simulink model "ceto"  (R2025a)
settings: Solver=ode4  StartTime=0  StopTime=200  FixedStep=0.01  MaxStep=0.01  RelTol=1e-3  EnableMultiTasking=on
values from neighbouring files (symbols this model uses):
  bemDepths = -3.0:-0.1:-15.0    [wecSimInputFile.m]
  PTO_motion_amplitude = 6    [wecSimInputFile.m]
  PTO_motion_period = 10    [createMCRMat.m]    (also in wecSimInputFile.m)
undefined symbols (not defined in the file or in its folder): body, pto
libraries: WECSim_Lib_Body_Elements x1, WECSim_Lib_Frames x1, WECSim_Lib_PTOs x1
settings Model: Creator=mlawson  LastModifiedBy=akeeste
settings SolverCC: ZeroCrossControl=DisableAll  AlgebraicLoopSolver=LineSearch  AutoInsertRateTranBlk=on
settings DataIOCC: SaveFormat=Array  SaveOutput=off  SaveTime=off  ReturnWorkspaceOutputs=off
settings OptimizationCC: LifeSpan=inf  SimCompilerOptimization=on
settings DebuggingCC: MergeDetectMultiDrivingBlocksExec=none  SolverPrmCheckMsg=warning  UnconnectedInputMsg=warning  UnconnectedOutputMsg=warning  UnconnectedLineMsg=warning  AllowSymbolicDim=off  StateNameClashWarn=warning  SFUnexpectedBacktrackingDiag=warning  SFNoUnconditionalDefaultTransitionDiag=warning  SFExecutionAtInitializationDiag=none  ArithmeticOperatorsInVariantConditions=warning
settings HardwareCC: ProdBitPerPointer=32.0  ProdBitPerSizeT=32.0  ProdBitPerPtrDiffT=32.0  ProdLargestAtomicFloat=None  ProdIntDivRoundTo=Undefined  ProdEndianess=Unspecified  ProdWordSize=32.0  ProdHWDeviceType=32-bit Generic
settings ModelReferenceCC: EnableRefExpFcnMdlSchedulingChecks=on  PropagateSignalLabelsOutOfModel=off
settings SFSimCC: SimUseLocalCustomCode=off  CustomCodeUndefinedFunction=UseInterfaceOnly
settings RTWCC: RTWUseLocalCustomCode=off  GPUComputeCapability=3.5  DLArmComputeVersion=19.05
settings CodeAppCC: StateflowObjectComments=on
settings GRTTargetCC: TargetLangStandard=C89/C90 (ANSI)
settings ConfigComp: CovMetricSettings=dw  CovSaveCumulativeToWorkspaceVar=on  CovSaveSingleToWorkspaceVar=on  CovExternalEMLEnable=off  CovSFcnEnable=off
settings SimscapeCC: SimscapeNormalizeSystem=off
settings ConfigurationSet: Description=SimMechanics 2G
settings ExplorerConfigSet: InternalSimMechanicsExplorerSettings="<ExplorerConfiguration><canonicalview>default</canonicalview><TilePanel><TileInfo><Tiles Columns=\"1\" Count=\"1\" Rows=\"1\"><Column Left=\"2\" Weight=\"1\"/><Column Left=\"1335\"/><Row Top=\"2\" Weight=\"1\"/><Row Top=\"911\"/><Tile Height=\"1\" Width=\"1\" X=\"0\" Y=\"0\"/></Tiles></TileInfo><SceneInfo><SceneViewer><BGColor><R>0.60000002384185791</R><G>0.60000002384185791</G><B>0.60000002384185791</B></BGColor><Camera><Position><X>365.37645888990272</X><Y>-369.82486814446582</Y><Z>359.64809521743916</Z></Position><Center><X>-6.7351450971904585</X><Y>2.2867358426280204</Y><Z>-12.463508769654169</Z></Center><Up><X>-0.40824829046386307</X><Y>0.40824829046386307</Y><Z>0.81649658092772615</Z></Up><Left>-57.820127362122818</Left><Right>57.820127362122818</Right><Bottom>-38.308817187253304</Bottom><Top>38.308817187253304</Top></Camera></SceneViewer></SceneInfo></TilePanel></ExplorerConfiguration>"

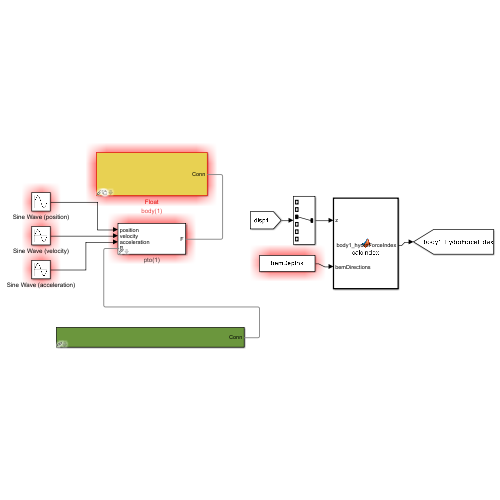
[thumbnail: Simulink's stored preview of the top-level diagram]
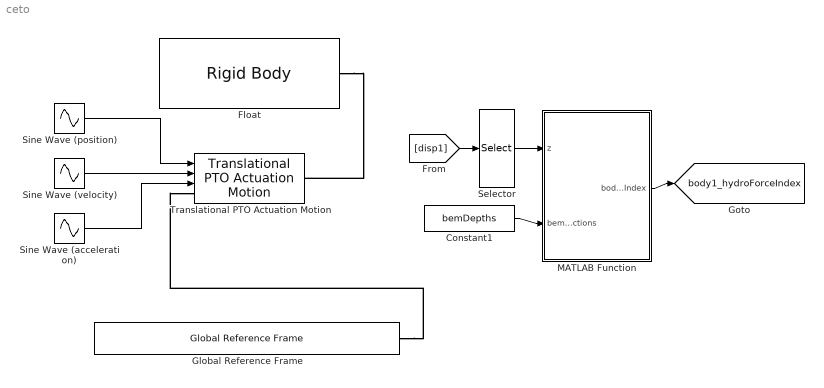
== system ceto ==
  Constant1 : Constant  Value=bemDepths
  Float : WECSim_Lib_Body_Elements/Rigid Body  body=body(1)
  Global Reference Frame : WECSim_Lib_Frames/Global Reference Frame  waves=waves  simu=simu
      settings: SourceProductName=WEC-Sim
  MATLAB Function : MATLAB Function  TreatAsAtomicUnit=on
  Selector : Selector  InputPortWidth=6  IndexOptions=Index vector (dialog)  Indices=[3]  OutputSizes=1
  Sine Wave (acceleration) : Sin  Amplitude=PTO_motion_amplitude*(2*pi / PTO_motion_period)^2  Frequency=(2*pi / PTO_motion_period)  Phase=pi  SampleTime=0
  Sine Wave (position) : Sin  Amplitude=PTO_motion_amplitude  Frequency=(2*pi / PTO_motion_period)  SampleTime=0
  Sine Wave (velocity) : Sin  Amplitude=PTO_motion_amplitude*(2*pi / PTO_motion_period)  Frequency=(2*pi / PTO_motion_period)  Phase=pi/2  SampleTime=0
  Translational PTO Actuation Motion : WECSim_Lib_PTOs/Translational PTO Actuation Motion  pto=pto(1)
      settings: AttributesFormatString=%<pto>
  tag scope: body1_hydroForceIndex=global
  wires:
  Sine Wave (position)/1 -> Translational PTO Actuation Motion/1
  Sine Wave (velocity)/1 -> Translational PTO Actuation Motion/2
  Sine Wave (acceleration)/1 -> Translational PTO Actuation Motion/3
  Constant1/1 -> MATLAB Function/2(bemDirections)
  MATLAB Function/1(body1_hydroForceIndex) -> [body1_hydroForceIndex]
  [disp1] -> Selector/1
  Selector/1 -> MATLAB Function/1(z)
  connections:
  Global Reference Frame/RConn1 -- Translational PTO Actuation Motion/LConn1
  Float/RConn1 -- Translational PTO Actuation Motion/RConn1

== matlab function ceto/MATLAB Function ==
  data: z input; bemDirections input; body1_hydroForceIndex output
function body1_hydroForceIndex  = calcIndex(z, bemDirections)

body1_hydroForceIndex  = calcIndex(z, bemDirections);

end
